simulink model "EMT_ML.before_diagnostic_fixes"  (R2024b)
settings: Solver=ode5  StartTime=0.0  StopTime=200  FixedStep=0.002  RelTol=1e-3
model workspace (MAT data in the model file):
  A = 7.3
  B = 2.71
  C0_shift = 200
  C1_shift = 200
  C2_shift = 200
  Cb = 70
  Cd = 0.6
  EMSInputBus : Simulink.Bus (value not decoded)
  Fb_max = 247500
  JA = 0.4
  JB = 0.4
  JZ = 0.4
  Jc1r2 = 0.01
  Jc3r4 = 0.01
  Jc4 = 0.01
  Je = 2.5
  Jh = 0.01
  Jq1 = 0.01
  Jq2 = 0.01
  Jr1 = 0.01
  Jr3s4 = 0.01
  Js123 = 0.01
  L = 4.472
  NE = [1600 1600 1600 1600 1600 1600 1600 1600 1600 1600 1600 1600 ... (840 elements, 30x28)]
  N_Te = 30
  N_ne = 28
  PE = [0 100.366530527 133.710336161 167.221698607 195.706356687 221.845219395 250.497434286 278.144308305 305.288511886 330.086920096 352.87464656 374.489475338 ... (840 elements, 30x28)]
  PN0 = 0
  Pb_epr = [-45 -45 -40 -30 0 30 40 45 45]
  Pb_max = [0 40 45 45 45]
  Pb_min = [-45 -45 -45 -40 0]
  Pe_ass = 230
  Pe_max = 1103
  Peg = [0 100 120 140 160 180 200 220 240 260 280 300 ... (53 elements, 1x53)]
  R_map = [0.09 0.089 0.09 0.091 0.092 0.093 0.094 0.095 0.096 0.097 0.098]
  SF_C0 = 1.5
  SF_C1 = 1.5
  SF_C2 = 1.5
  SF_Z1 = 1.5
  SF_Z2 = 1.5
  SF_ZD = 1.5
  SOC0 = 60
  SOC_epr = [30 31 50 59 60 61 70 79 80]
  SOC_map = [0 10 20 30 40 50 60 70 80 90 100]
  TA_max_map = [588.855 593.803361345 598.83559322 603.953846154 609.160344828 614.457391304 619.847368421 625.332743363 630.916071429 636.6 642.387272727 648.280733945 ... (115 elements, 1x115)]
  TA_min_map = [-588.855 -593.803361345 -598.83559322 -603.953846154 -609.160344828 -614.457391304 -619.847368421 -625.332743363 -630.916071429 -636.6 -642.387272727 -648.280733945 ... (115 elements, 1x115)]
  TAf = 0
  TB_max_map = [588.855 593.803361345 598.83559322 603.953846154 609.160344828 614.457391304 619.847368421 625.332743363 630.916071429 636.6 642.387272727 648.280733945 ... (115 elements, 1x115)]
  TB_min_map = [-588.855 -593.803361345 -598.83559322 -603.953846154 -609.160344828 -614.457391304 -619.847368421 -625.332743363 -630.916071429 -636.6 -642.387272727 -648.280733945 ... (115 elements, 1x115)]
  TBf = 0
  TE = [0 599 798 998 1168 1324 1495 1660 1822 1970 2106 2235 ... (840 elements, 30x28)]
  TS_A = 0.2
  TS_B = 0.2
  TS_C0 = 0.2
  TS_C1 = 0.2
  TS_C2 = 0.2
  TS_Z = 0.2
  TS_Z1 = 0.2
  TS_Z2 = 0.2
  TS_ZD = 0.2
  TZ_max_map = [537.13125 540.509433962 543.930379747 547.394904459 550.903846154 554.458064516 558.058441558 561.705882353 565.401315789 569.145695364 572.94 576.785234899 ... (131 elements, 1x131)]
  TZ_min_map = [-537.13125 -540.509433962 -543.930379747 -547.394904459 -550.903846154 -554.458064516 -558.058441558 -561.705882353 -565.401315789 -569.145695364 -572.94 -576.785234899 ... (131 elements, 1x131)]
  TZf = 0
  T_generator = [0 185 493.333333333 801.666666667 1110 1418.33333333 1726.66666667]
  T_motor = [0 185 493.333333333 801.666666667 1110 1418.33333333 1726.66666667]
  Te_map = [0 599 798 998 1168 1324 1495 1660 1822 1970 2106 2235 ... (30 elements, 1x30)]
  Te_max = 2754
  Te_max_map = [1168 1324 1495 1660 1822 1970 2106 2235 2355 2458 2543 2606 ... (28 elements, 1x28)]
  Te_start = 1600
  Tef = 100
  Teg = [0 596.8125 636.6 718.741935484 799.916230366 859.41 954.422788606 954.9 996.417391304 1078.98305085 1114.05 1169.26530612 ... (53 elements, 1x53)]
  Temax = 998
  Time = [0 0.1 0.2 0.3 0.4 0.5 0.6 0.7 0.8 0.9 1 1.1 ... (2001 elements, 1x2001)]
  Time_ele = [0 4 8 12 16 20 24 28 32 36 40 44 ... (401 elements, 1x401)]
  Time_fg = [0 2 4 6 8 10 12 14 16 18 20 22 ... (801 elements, 1x801)]
  Tmax_C0 = 2754
  Tmax_C1 = 3505.25455609
  Tmax_C2 = 3505.25455609
  Tmax_Z1 = 5584.80955498
  Tmax_Z2 = 16307.6439005
  Tmax_ZD = 3855.6
  Ts_e = 0.1
  Uoc_map = [814.5 917 933.25 945.75 958.25 969.25 978 985.25 993.25 1003.25 1050]
  V_Shift12 = 32
  V_Shift21 = 25
  V_Start = 10
  Voltage0 = 900
  Voltage_epr = [750 760 900 1000 1050]
  Y_engine = 0.955
  Yc = 0.98
  Yh = 0.96
  Yo = 0.92
  Yq = 0.94
  Z1_shift = 200
  Z2_shift = 200
  a11 = 1.54241568346
  a11_L = 1.54241568346
  a12 = -3.86074191629
  a12_L = 2.43173643789
  a21 = -1.04963112005
  a22 = 2.46948356808
  b11 = 0
  b11_L = 0
  b12 = 3.33
  b12_L = 7.8036
  b21 = 2.23571428571
  b22 = -2.13
  c11 = -0.648333656565
  c12 = 0
  c21 = -0.648333656565
  c22 = 0.680511182109
  controller_id = 1
  controller_name = 'Existing heuristic-grid EMS'
  cycle_grade = [0 0 0 0 0 0 0 0 0 0 0 0 ... (2001 elements, 1x2001)]
  cycle_road = [0.045 0.045 0.045 0.045 0.045 0.045 0.045 0.045 0.045 0.045 0.045 0.045 ... (2001 elements, 1x2001)]
  cycle_steering = [0 0 0 0 0 0 0 0 0 0 0 0 ... (2001 elements, 1x2001)]
  cycle_time = [0 0.1 0.2 0.3 0.4 0.5 0.6 0.7 0.8 0.9 1 1.1 ... (2001 elements, 1x2001)]
  d11 = -0.751666343435
  d12 = 0.3003003003
  d21 = -0.751666343435
  d22 = 0.319488817891
  e11 = -1.54241568346
  e12 = 0
  e21 = 1.04963112005
  e22 = -2.23571428571
  eff_generator = [0.8 0.8 0.79 0.79 0.76 0.74 0.72 0.8 0.85 0.88 0.85 0.8 ... (84 elements, 7x12)]
  eff_motor = [0.8 0.8 0.79 0.79 0.76 0.74 0.72 0.8 0.85 0.88 0.85 0.8 ... (84 elements, 7x12)]
  ele_map = [10 11.46 14.13 19.24 20.94 23.21 20.29 20.23 22.28 17.66 16.24 18.95 ... (401 elements, 1x401)]
  ems_runtime_config : object (value not decoded)
  f11 = -3.86074191629
  f12 = 3.33
  f21 = 2.46948356808
  f22 = -2.13
  fg = 0.045
  fg_map = [0.0125 0.0215 0.0332 0.0452 0.0525 0.0589 0.0584 0.0592 0.0621 0.0576 0.055 0.0572 ... (801 elements, 1x801)]
  fuel_gpkwh = [269.874826377 269.874826377 260.084605263 254.895150301 249.802821062 244.062054381 234.972466555 226.630558735 223.93243551 227.612775381 231.379615385 228.983738255 ... (840 elements, 30x28)]
  fuel_map = [269.874826377 269.874826377 260.084605263 254.895150301 249.802821062 244.062054381 234.972466555 226.630558735 223.93243551 227.612775381 231.379615385 228.983738255 ... (840 elements, 30x28)]
  fuel_map_N = [269.874826377 269.874826377 260.084605263 254.895150301 249.802821062 nan nan nan nan nan nan nan ... (840 elements, 30x28)]
  i = 28
  ic = 4.42
  iq = 1.4
  it = 4
  j = 30
  k1 = 2.13
  k2 = 2.13
  k3 = 2.33
  k4 = 1.92
  kh = 2.88
  kq = 2.17
  kt = 1.83
  mass = 45000
  miu_max = 0.8
  nA_map = [-6000 -5950 -5900 -5850 -5800 -5750 -5700 -5650 -5600 -5550 -5500 -5450 ... (115 elements, 1x115)]
  nA_max = 6000
  nA_min = -6000
  nB_map = [-6000 -5950 -5900 -5850 -5800 -5750 -5700 -5650 -5600 -5550 -5500 -5450 ... (115 elements, 1x115)]
  nB_max = 6000
  nB_min = -6000
  nB_start = 0
  nZ_map = [-8000 -7950 -7900 -7850 -7800 -7750 -7700 -7650 -7600 -7550 -7500 -7450 ... (131 elements, 1x131)]
  nZ_max = 8000
  nZ_min = -8000
  n_generator = [0 318.5 796.25 1274 1751.75 2229.5 2707.25 3185 3662.75 4140.5 4618.25 7007]
  n_motor = [0 318.5 796.25 1274 1751.75 2229.5 2707.25 3185 3662.75 4140.5 4618.25 7007]
  ne_idl = 3000
  ne_map = [1600 1700 1800 1900 2000 2100 2200 2300 2400 2500 2600 2700 ... (28 elements, 1x28)]
  ne_max = 4200
  ne_min = 1600
  ne_start = 200
  neg = [1600 1600 1800 1860 1910 2000 2001 2200 2300 2301 2400 2450 ... (53 elements, 1x53)]
  no_Shift12 = 1589.43589002
  no_Shift21 = 1241.74678908
  rz = 0.318
  startup_feedback_delay_s = 0.002
  startup_power_share = 0.5
  startup_speed_regularizer_rpm = 100
  v_cyc = [0 0 0 0 0 0 0 0 0 0 0 0 ... (2001 elements, 1x2001)]
  voltage_HighA = 1050
  voltage_HighB = 1050
  voltage_HighZ = 1050
  voltage_LowA = 750
  voltage_LowB = 750
  voltage_LowZ = 750
symbols that are objects in the model workspace (value not decoded): ems_runtime_config
undefined symbols (not defined in the file or in its folder): sigbuilder_block
libraries: fl_lib x82, nesl_utility x55, simulink x49, sdl_lib x10, simulink_need_slupdate x6, powerlib_extras x1
(part 6 of 7)

== system EMT_ML.before_diagnostic_fixes/Control Unit/Control/Shift Stage/EVT2->EVT1/engine torque ==
  Te_com : Outport
  wires:
  [Te_ref] -> Te_com/1

== system EMT_ML.before_diagnostic_fixes/Control Unit/Control/Shift Stage/EVT2->EVT1/motorA torque ==
  TA_com : Outport
  wires:
  [TA_ref] -> TA_com/1

== system EMT_ML.before_diagnostic_fixes/Control Unit/Control/Shift Stage/EVT2->EVT1/motorB torque ==
  TB_com : Outport
  wires:
  [TB_ref] -> TB_com/1

== system EMT_ML.before_diagnostic_fixes/Control Unit/Control/Shift Stage/EVT2->EVT1/motorZ torque ==
  Lookup Table : Lookup  InputValues=nZ_map  Table=TZ_max_map  SaturateOnIntegerOverflow=off
  Lookup Table1 : Lookup  InputValues=nZ_map  Table=TZ_min_map  SaturateOnIntegerOverflow=off
  Saturation Dynamic : simulink/Discontinuities/Saturation Dynamic  OutMin=[]  OutMax=[]  OutDataTypeStr=Inherit: Same as second input  OutDataType=sfix(16)  OutScaling=2^-10  DoSatur=off
  Saturation1 : Saturate  UpperLimit=max(nZ_map)  LowerLimit=min(nZ_map)
  Saturation2 : Saturate  UpperLimit=max(nZ_map)  LowerLimit=min(nZ_map)
  Subsystem1 : Subsystem
  TZ_com : Outport
  wires:
  Saturation Dynamic/1 -> TZ_com/1
  [nZ_act] -> Saturation1/1, Saturation2/1, Subsystem1/1(nZ_act)
  Lookup Table/1 -> Saturation Dynamic/1
  Lookup Table1/1 -> Saturation Dynamic/3
  Saturation1/1 -> Lookup Table/1
  Saturation2/1 -> Lookup Table1/1
  Subsystem1/1(TZ_com) -> Saturation Dynamic/2

== system EMT_ML.before_diagnostic_fixes/Control Unit/Driver/Electric Power Requirement/Subsystem4/Subsystem4 ==
  11 : Constant
  21 : Constant  Value=2
  22 : Constant  Value=3
  31 : Constant  Value=4
  0.1 : Outport
  0.01 : Outport  Port=2
  10 : Outport  Port=3
  100 : Outport  Port=4
  wires:
  31/1 -> 100/1
  22/1 -> 10/1
  21/1 -> 0.01/1
  11/1 -> 0.1/1

== system EMT_ML.before_diagnostic_fixes/Control Unit/Driver/Electric Power Requirement/Subsystem4/Subsystem6 ==
  11 : Constant
  21 : Constant  Value=2
  22 : Constant  Value=3
  31 : Constant  Value=4
  1 : Outport
  2 : Outport  Port=2
  3 : Outport  Port=3
  4 : Outport  Port=4
  wires:
  11/1 -> 1/1
  21/1 -> 2/1
  22/1 -> 3/1
  31/1 -> 4/1

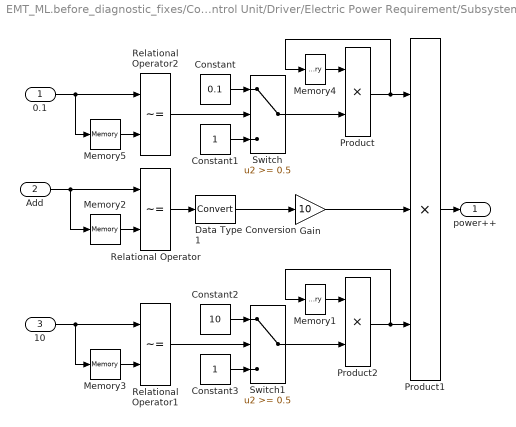
== system EMT_ML.before_diagnostic_fixes/Control Unit/Driver/Electric Power Requirement/Subsystem6/Subsystem ==
  0.1 : Inport
  Add : Inport  Port=2
  10 : Inport  Port=3
  Constant : Constant  Value=0.1
  Constant1 : Constant
  Constant2 : Constant  Value=10
  Constant3 : Constant
  Data Type Conversion1 : DataTypeConversion  SaturateOnIntegerOverflow=off  RndMeth=Floor
  Gain : Gain  Gain=10
  Memory1 : Memory  InitialCondition=1
  Memory2 : Memory
  Memory3 : Memory
  Memory4 : Memory  InitialCondition=1
  Memory5 : Memory
  Product : Product  RndMeth=Zero
  Product1 : Product  Inputs=3  RndMeth=Zero
  Product2 : Product  RndMeth=Zero
  Relational Operator : RelationalOperator  Operator=~=  OutDataTypeStr=boolean  InputSameDT=off
  Relational Operator1 : RelationalOperator  Operator=~=  OutDataTypeStr=boolean  InputSameDT=off
  Relational Operator2 : RelationalOperator  Operator=~=  OutDataTypeStr=boolean  InputSameDT=off
  Switch : Switch  Threshold=0.5  SaturateOnIntegerOverflow=off  InputSameDT=off
  Switch1 : Switch  Threshold=0.5  SaturateOnIntegerOverflow=off  InputSameDT=off
  power++ : Outport
  wires:
  Memory2/1 -> Relational Operator/2
  Add/1 -> Relational Operator/1, Memory2/1
  Relational Operator/1 -> Data Type Conversion1/1
  Data Type Conversion1/1 -> Gain/1
  Product/1 -> Memory4/1, Product1/1
  Memory4/1 -> Product/1
  Memory5/1 -> Relational Operator2/2
  Relational Operator2/1 -> Switch/2
  0.1/1 -> Memory5/1, Relational Operator2/1
  Constant/1 -> Switch/1
  Constant1/1 -> Switch/3
  Switch/1 -> Product/2
  Product1/1 -> power++/1
  Product2/1 -> Memory1/1, Product1/3
  Memory1/1 -> Product2/1
  Memory3/1 -> Relational Operator1/2
  Relational Operator1/1 -> Switch1/2
  10/1 -> Relational Operator1/1, Memory3/1
  Constant2/1 -> Switch1/1
  Constant3/1 -> Switch1/3
  Switch1/1 -> Product2/2
  Gain/1 -> Product1/2

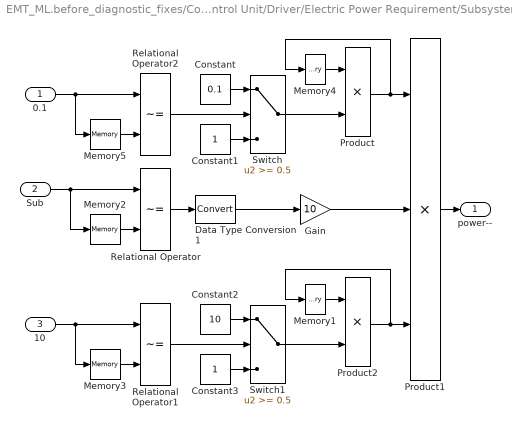
== system EMT_ML.before_diagnostic_fixes/Control Unit/Driver/Electric Power Requirement/Subsystem6/Subsystem1 ==
  0.1 : Inport
  Sub : Inport  Port=2
  10 : Inport  Port=3
  Constant : Constant  Value=0.1
  Constant1 : Constant
  Constant2 : Constant  Value=10
  Constant3 : Constant
  Data Type Conversion1 : DataTypeConversion  SaturateOnIntegerOverflow=off  RndMeth=Floor
  Gain : Gain  Gain=10
  Memory1 : Memory  InitialCondition=1
  Memory2 : Memory
  Memory3 : Memory
  Memory4 : Memory  InitialCondition=1
  Memory5 : Memory
  Product : Product  RndMeth=Zero
  Product1 : Product  Inputs=3  RndMeth=Zero
  Product2 : Product  RndMeth=Zero
  Relational Operator : RelationalOperator  Operator=~=  OutDataTypeStr=boolean  InputSameDT=off
  Relational Operator1 : RelationalOperator  Operator=~=  OutDataTypeStr=boolean  InputSameDT=off
  Relational Operator2 : RelationalOperator  Operator=~=  OutDataTypeStr=boolean  InputSameDT=off
  Switch : Switch  Threshold=0.5  SaturateOnIntegerOverflow=off  InputSameDT=off
  Switch1 : Switch  Threshold=0.5  SaturateOnIntegerOverflow=off  InputSameDT=off
  power-- : Outport
  wires:
  Switch1/1 -> Product2/2
  Constant3/1 -> Switch1/3
  Constant2/1 -> Switch1/1
  10/1 -> Memory3/1, Relational Operator1/1
  Relational Operator1/1 -> Switch1/2
  Memory3/1 -> Relational Operator1/2
  Memory1/1 -> Product2/1
  Product2/1 -> Product1/3, Memory1/1
  Product1/1 -> power--/1
  Switch/1 -> Product/2
  Constant1/1 -> Switch/3
  Constant/1 -> Switch/1
  0.1/1 -> Relational Operator2/1, Memory5/1
  Relational Operator2/1 -> Switch/2
  Memory5/1 -> Relational Operator2/2
  Memory4/1 -> Product/1
  Product/1 -> Product1/1, Memory4/1
  Data Type Conversion1/1 -> Gain/1
  Relational Operator/1 -> Data Type Conversion1/1
  Sub/1 -> Memory2/1, Relational Operator/1
  Memory2/1 -> Relational Operator/2
  Gain/1 -> Product1/2

== system EMT_ML.before_diagnostic_fixes/Control Unit/Driver/Grade Angle/Subsystem4/Subsystem4 ==
  11 : Constant
  21 : Constant  Value=2
  22 : Constant  Value=3
  31 : Constant  Value=4
  0.1 : Outport
  0.01 : Outport  Port=2
  10 : Outport  Port=3
  100 : Outport  Port=4
  wires:
  31/1 -> 100/1
  22/1 -> 10/1
  21/1 -> 0.01/1
  11/1 -> 0.1/1

== system EMT_ML.before_diagnostic_fixes/Control Unit/Driver/Grade Angle/Subsystem4/Subsystem6 ==
  11 : Constant
  21 : Constant  Value=2
  22 : Constant  Value=3
  31 : Constant  Value=4
  1 : Outport
  2 : Outport  Port=2
  3 : Outport  Port=3
  4 : Outport  Port=4
  wires:
  11/1 -> 1/1
  21/1 -> 2/1
  22/1 -> 3/1
  31/1 -> 4/1

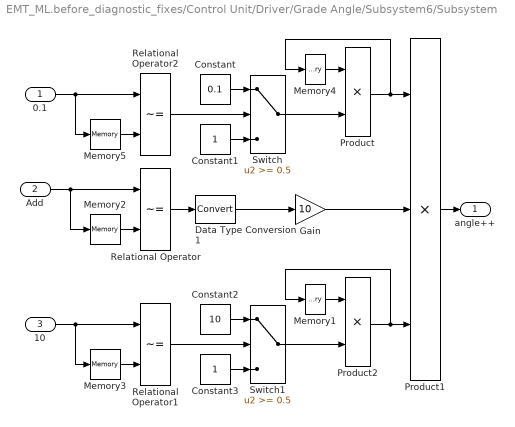
== system EMT_ML.before_diagnostic_fixes/Control Unit/Driver/Grade Angle/Subsystem6/Subsystem ==
  0.1 : Inport
  Add : Inport  Port=2
  10 : Inport  Port=3
  Constant : Constant  Value=0.1
  Constant1 : Constant
  Constant2 : Constant  Value=10
  Constant3 : Constant
  Data Type Conversion1 : DataTypeConversion  SaturateOnIntegerOverflow=off  RndMeth=Floor
  Gain : Gain  Gain=10
  Memory1 : Memory  InitialCondition=1
  Memory2 : Memory
  Memory3 : Memory
  Memory4 : Memory  InitialCondition=1
  Memory5 : Memory
  Product : Product  RndMeth=Zero
  Product1 : Product  Inputs=3  RndMeth=Zero
  Product2 : Product  RndMeth=Zero
  Relational Operator : RelationalOperator  Operator=~=  OutDataTypeStr=boolean  InputSameDT=off
  Relational Operator1 : RelationalOperator  Operator=~=  OutDataTypeStr=boolean  InputSameDT=off
  Relational Operator2 : RelationalOperator  Operator=~=  OutDataTypeStr=boolean  InputSameDT=off
  Switch : Switch  Threshold=0.5  SaturateOnIntegerOverflow=off  InputSameDT=off
  Switch1 : Switch  Threshold=0.5  SaturateOnIntegerOverflow=off  InputSameDT=off
  angle++ : Outport
  wires:
  Memory2/1 -> Relational Operator/2
  Add/1 -> Relational Operator/1, Memory2/1
  Relational Operator/1 -> Data Type Conversion1/1
  Data Type Conversion1/1 -> Gain/1
  Product/1 -> Memory4/1, Product1/1
  Memory4/1 -> Product/1
  Memory5/1 -> Relational Operator2/2
  Relational Operator2/1 -> Switch/2
  0.1/1 -> Memory5/1, Relational Operator2/1
  Constant/1 -> Switch/1
  Constant1/1 -> Switch/3
  Switch/1 -> Product/2
  Product1/1 -> angle++/1
  Product2/1 -> Memory1/1, Product1/3
  Memory1/1 -> Product2/1
  Memory3/1 -> Relational Operator1/2
  Relational Operator1/1 -> Switch1/2
  10/1 -> Relational Operator1/1, Memory3/1
  Constant2/1 -> Switch1/1
  Constant3/1 -> Switch1/3
  Switch1/1 -> Product2/2
  Gain/1 -> Product1/2

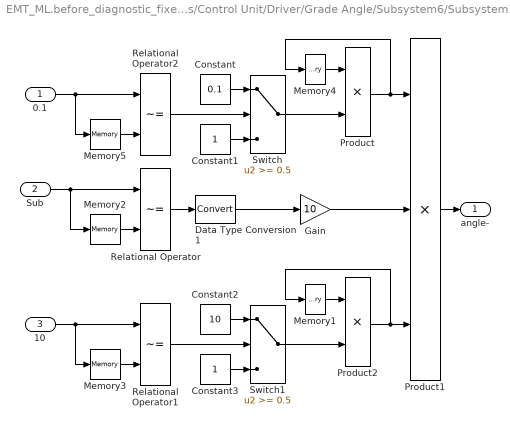
== system EMT_ML.before_diagnostic_fixes/Control Unit/Driver/Grade Angle/Subsystem6/Subsystem1 ==
  0.1 : Inport
  Sub : Inport  Port=2
  10 : Inport  Port=3
  Constant : Constant  Value=0.1
  Constant1 : Constant
  Constant2 : Constant  Value=10
  Constant3 : Constant
  Data Type Conversion1 : DataTypeConversion  SaturateOnIntegerOverflow=off  RndMeth=Floor
  Gain : Gain  Gain=10
  Memory1 : Memory  InitialCondition=1
  Memory2 : Memory
  Memory3 : Memory
  Memory4 : Memory  InitialCondition=1
  Memory5 : Memory
  Product : Product  RndMeth=Zero
  Product1 : Product  Inputs=3  RndMeth=Zero
  Product2 : Product  RndMeth=Zero
  Relational Operator : RelationalOperator  Operator=~=  OutDataTypeStr=boolean  InputSameDT=off
  Relational Operator1 : RelationalOperator  Operator=~=  OutDataTypeStr=boolean  InputSameDT=off
  Relational Operator2 : RelationalOperator  Operator=~=  OutDataTypeStr=boolean  InputSameDT=off
  Switch : Switch  Threshold=0.5  SaturateOnIntegerOverflow=off  InputSameDT=off
  Switch1 : Switch  Threshold=0.5  SaturateOnIntegerOverflow=off  InputSameDT=off
  angle- : Outport
  wires:
  Switch1/1 -> Product2/2
  Constant3/1 -> Switch1/3
  Constant2/1 -> Switch1/1
  10/1 -> Memory3/1, Relational Operator1/1
  Relational Operator1/1 -> Switch1/2
  Memory3/1 -> Relational Operator1/2
  Memory1/1 -> Product2/1
  Product2/1 -> Product1/3, Memory1/1
  Product1/1 -> angle-/1
  Switch/1 -> Product/2
  Constant1/1 -> Switch/3
  Constant/1 -> Switch/1
  0.1/1 -> Relational Operator2/1, Memory5/1
  Relational Operator2/1 -> Switch/2
  Memory5/1 -> Relational Operator2/2
  Memory4/1 -> Product/1
  Product/1 -> Product1/1, Memory4/1
  Data Type Conversion1/1 -> Gain/1
  Relational Operator/1 -> Data Type Conversion1/1
  Sub/1 -> Memory2/1, Relational Operator/1
  Memory2/1 -> Relational Operator/2
  Gain/1 -> Product1/2

== system EMT_ML.before_diagnostic_fixes/Control Unit/Driver/Ground Resistance Coefficient/Road/Subsystem ==
  In : Inport
  Add : Sum  Inputs=+++
  Compare To Constant1 : simulink/Logic and Bit Operations/Compare To Constant  relop=>  const=0.01  OutDataTypeStr=uint8
  Compare To Constant2 : simulink/Logic and Bit Operations/Compare To Constant  relop=>  const=0.2  OutDataTypeStr=uint8
  Compare To Constant3 : simulink/Logic and Bit Operations/Compare To Constant  relop=>  const=0.8  OutDataTypeStr=uint8
  Compare To Constant4 : simulink/Logic and Bit Operations/Compare To Constant  relop=<  const=1  OutDataTypeStr=uint8
  Data Type Conversion : DataTypeConversion  SaturateOnIntegerOverflow=off  RndMeth=Floor
  Logical Operator1 : Logic  Operator=OR  AllPortsSameDT=off  OutDataTypeStr=boolean
  Memory2 : Memory
  Judge : Outport
  wires:
  Compare To Constant2/1 -> Add/2
  Data Type Conversion/1 -> Judge/1
  Compare To Constant1/1 -> Add/1
  Add/1 -> Data Type Conversion/1
  In/1 -> Compare To Constant3/1, Compare To Constant2/1, Compare To Constant1/1
  [v_act] -> Memory2/1
  Memory2/1 -> Compare To Constant4/1
  Compare To Constant4/1 -> Logical Operator1/2
  Compare To Constant3/1 -> Logical Operator1/1
  Logical Operator1/1 -> Add/3

== system EMT_ML.before_diagnostic_fixes/Control Unit/Driver/Ground Resistance Coefficient/Road/Subsystem1 ==
  Constant5 : Constant  Value=0.6
  Out1 : Outport
  wires:
  Constant5/1 -> Out1/1

== system EMT_ML.before_diagnostic_fixes/Control Unit/Driver/Ground Resistance Coefficient/Road/Subsystem2 ==
  In1 : Inport
  1-D Lookup Table : Lookup_n-D  NumberOfTableDimensions=1  BreakpointsForDimension1=[-1 0 0.1 0.2 0.8 1]  Table=[0.6 0.1 0.04 0 0 0]  RndMeth=Simplest
  Saturation : Saturate  UpperLimit=1  LowerLimit=-1
  Out1 : Outport
  wires:
  Saturation/1 -> 1-D Lookup Table/1
  In1/1 -> Saturation/1
  1-D Lookup Table/1 -> Out1/1

== system EMT_ML.before_diagnostic_fixes/Control Unit/Driver/Ground Resistance Coefficient/Road/Subsystem3 ==
  Constant1 : Constant  Value=0
  Out1 : Outport
  wires:
  Constant1/1 -> Out1/1

== system EMT_ML.before_diagnostic_fixes/Control Unit/Driver/Ground Resistance Coefficient/Road/Subsystem4 ==
  Constant1 : Constant  Value=-0.04
  Out1 : Outport
  wires:
  Constant1/1 -> Out1/1

== system EMT_ML.before_diagnostic_fixes/Control Unit/Driver/Ground Resistance Coefficient/Subsystem2/Subsystem4 ==
  11 : Constant
  21 : Constant  Value=2
  22 : Constant  Value=3
  31 : Constant  Value=4
  0.1 : Outport
  0.01 : Outport  Port=2
  10 : Outport  Port=3
  100 : Outport  Port=4
  wires:
  11/1 -> 0.1/1
  21/1 -> 0.01/1
  22/1 -> 10/1
  31/1 -> 100/1

== system EMT_ML.before_diagnostic_fixes/Control Unit/Driver/Ground Resistance Coefficient/Subsystem2/Subsystem6 ==
  11 : Constant
  21 : Constant  Value=2
  22 : Constant  Value=3
  31 : Constant  Value=4
  1 : Outport
  2 : Outport  Port=2
  3 : Outport  Port=3
  4 : Outport  Port=4
  wires:
  31/1 -> 4/1
  22/1 -> 3/1
  21/1 -> 2/1
  11/1 -> 1/1

== system EMT_ML.before_diagnostic_fixes/Control Unit/Driver/Ground Resistance Coefficient/Subsystem3/Subsystem ==
  0.1 : Inport
  Add : Inport  Port=2
  10 : Inport  Port=3
  Constant : Constant  Value=0.1
  Constant1 : Constant
  Constant2 : Constant  Value=10
  Constant3 : Constant
  Data Type Conversion1 : DataTypeConversion  SaturateOnIntegerOverflow=off  RndMeth=Floor
  Gain : Gain  Gain=0.01
  Memory1 : Memory  InitialCondition=1
  Memory2 : Memory
  Memory3 : Memory
  Memory4 : Memory  InitialCondition=1
  Memory5 : Memory
  Product : Product  RndMeth=Zero
  Product1 : Product  Inputs=3  RndMeth=Zero
  Product2 : Product  RndMeth=Zero
  Relational Operator : RelationalOperator  Operator=~=  OutDataTypeStr=boolean  InputSameDT=off
  Relational Operator1 : RelationalOperator  Operator=~=  OutDataTypeStr=boolean  InputSameDT=off
  Relational Operator2 : RelationalOperator  Operator=~=  OutDataTypeStr=boolean  InputSameDT=off
  Switch : Switch  Threshold=0.5  SaturateOnIntegerOverflow=off  InputSameDT=off
  Switch1 : Switch  Threshold=0.5  SaturateOnIntegerOverflow=off  InputSameDT=off
  fg++ : Outport
  wires:
  Gain/1 -> Product1/2
  Switch1/1 -> Product2/2
  Constant3/1 -> Switch1/3
  Constant2/1 -> Switch1/1
  10/1 -> Memory3/1, Relational Operator1/1
  Relational Operator1/1 -> Switch1/2
  Memory3/1 -> Relational Operator1/2
  Memory1/1 -> Product2/1
  Product2/1 -> Product1/3, Memory1/1
  Product1/1 -> fg++/1
  Switch/1 -> Product/2
  Constant1/1 -> Switch/3
  Constant/1 -> Switch/1
  0.1/1 -> Relational Operator2/1, Memory5/1
  Relational Operator2/1 -> Switch/2
  Memory5/1 -> Relational Operator2/2
  Memory4/1 -> Product/1
  Product/1 -> Product1/1, Memory4/1
  Data Type Conversion1/1 -> Gain/1
  Relational Operator/1 -> Data Type Conversion1/1
  Add/1 -> Memory2/1, Relational Operator/1
  Memory2/1 -> Relational Operator/2

== system EMT_ML.before_diagnostic_fixes/Control Unit/Driver/Ground Resistance Coefficient/Subsystem3/Subsystem1 ==
  0.1 : Inport
  Sub : Inport  Port=2
  10 : Inport  Port=3
  Constant : Constant  Value=0.1
  Constant1 : Constant
  Constant2 : Constant  Value=10
  Constant3 : Constant
  Data Type Conversion1 : DataTypeConversion  SaturateOnIntegerOverflow=off  RndMeth=Floor
  Gain : Gain  Gain=0.01
  Memory1 : Memory  InitialCondition=1
  Memory2 : Memory
  Memory3 : Memory
  Memory4 : Memory  InitialCondition=1
  Memory5 : Memory
  Product : Product  RndMeth=Zero
  Product1 : Product  Inputs=3  RndMeth=Zero
  Product2 : Product  RndMeth=Zero
  Relational Operator : RelationalOperator  Operator=~=  OutDataTypeStr=boolean  InputSameDT=off
  Relational Operator1 : RelationalOperator  Operator=~=  OutDataTypeStr=boolean  InputSameDT=off
  Relational Operator2 : RelationalOperator  Operator=~=  OutDataTypeStr=boolean  InputSameDT=off
  Switch : Switch  Threshold=0.5  SaturateOnIntegerOverflow=off  InputSameDT=off
  Switch1 : Switch  Threshold=0.5  SaturateOnIntegerOverflow=off  InputSameDT=off
  fg-- : Outport
  wires:
  Gain/1 -> Product1/2
  Memory2/1 -> Relational Operator/2
  Sub/1 -> Relational Operator/1, Memory2/1
  Relational Operator/1 -> Data Type Conversion1/1
  Data Type Conversion1/1 -> Gain/1
  Product/1 -> Memory4/1, Product1/1
  Memory4/1 -> Product/1
  Memory5/1 -> Relational Operator2/2
  Relational Operator2/1 -> Switch/2
  0.1/1 -> Memory5/1, Relational Operator2/1
  Constant/1 -> Switch/1
  Constant1/1 -> Switch/3
  Switch/1 -> Product/2
  Product1/1 -> fg--/1
  Product2/1 -> Memory1/1, Product1/3
  Memory1/1 -> Product2/1
  Memory3/1 -> Relational Operator1/2
  Relational Operator1/1 -> Switch1/2
  10/1 -> Relational Operator1/1, Memory3/1
  Constant2/1 -> Switch1/1
  Constant3/1 -> Switch1/3
  Switch1/1 -> Product2/2

== system EMT_ML.before_diagnostic_fixes/Control Unit/Driver/Pedal /Subsystem13/Subsystem4 ==
  11 : Constant
  21 : Constant  Value=2
  22 : Constant  Value=3
  31 : Constant  Value=4
  0.1 : Outport
  0.01 : Outport  Port=2
  10 : Outport  Port=3
  100 : Outport  Port=4
  wires:
  31/1 -> 100/1
  22/1 -> 10/1
  21/1 -> 0.01/1
  11/1 -> 0.1/1

== system EMT_ML.before_diagnostic_fixes/Control Unit/Driver/Pedal /Subsystem13/Subsystem6 ==
  11 : Constant
  21 : Constant  Value=2
  22 : Constant  Value=3
  31 : Constant  Value=4
  1 : Outport
  2 : Outport  Port=2
  3 : Outport  Port=3
  4 : Outport  Port=4
  wires:
  11/1 -> 1/1
  21/1 -> 2/1
  22/1 -> 3/1
  31/1 -> 4/1

== system EMT_ML.before_diagnostic_fixes/Control Unit/Driver/Pedal /Subsystem5/Subsystem ==
  0.1 : Inport
  Add : Inport  Port=2
  10 : Inport  Port=3
  Constant : Constant  Value=0.1
  Constant1 : Constant
  Constant2 : Constant  Value=10
  Constant3 : Constant
  Data Type Conversion1 : DataTypeConversion  SaturateOnIntegerOverflow=off  RndMeth=Floor
  Gain : Gain  Gain=0.1
  Memory1 : Memory  InitialCondition=1
  Memory2 : Memory
  Memory3 : Memory
  Memory4 : Memory  InitialCondition=1
  Memory5 : Memory
  Product : Product  RndMeth=Zero
  Product1 : Product  Inputs=3  RndMeth=Zero
  Product2 : Product  RndMeth=Zero
  Relational Operator : RelationalOperator  Operator=~=  OutDataTypeStr=boolean  InputSameDT=off
  Relational Operator1 : RelationalOperator  Operator=~=  OutDataTypeStr=boolean  InputSameDT=off
  Relational Operator2 : RelationalOperator  Operator=~=  OutDataTypeStr=boolean  InputSameDT=off
  Switch : Switch  Threshold=0.5  SaturateOnIntegerOverflow=off  InputSameDT=off
  Switch1 : Switch  Threshold=0.5  SaturateOnIntegerOverflow=off  InputSameDT=off
  pedal++ : Outport
  wires:
  Memory2/1 -> Relational Operator/2
  Add/1 -> Relational Operator/1, Memory2/1
  Relational Operator/1 -> Data Type Conversion1/1
  Data Type Conversion1/1 -> Gain/1
  Product/1 -> Memory4/1, Product1/1
  Memory4/1 -> Product/1
  Memory5/1 -> Relational Operator2/2
  Relational Operator2/1 -> Switch/2
  0.1/1 -> Memory5/1, Relational Operator2/1
  Constant/1 -> Switch/1
  Constant1/1 -> Switch/3
  Switch/1 -> Product/2
  Product1/1 -> pedal++/1
  Product2/1 -> Memory1/1, Product1/3
  Memory1/1 -> Product2/1
  Memory3/1 -> Relational Operator1/2
  Relational Operator1/1 -> Switch1/2
  10/1 -> Relational Operator1/1, Memory3/1
  Constant2/1 -> Switch1/1
  Constant3/1 -> Switch1/3
  Switch1/1 -> Product2/2
  Gain/1 -> Product1/2

== system EMT_ML.before_diagnostic_fixes/Control Unit/Driver/Pedal /Subsystem5/Subsystem1 ==
  0.1 : Inport
  Sub : Inport  Port=2
  10 : Inport  Port=3
  Constant : Constant  Value=0.1
  Constant1 : Constant
  Constant2 : Constant  Value=10
  Constant3 : Constant
  Data Type Conversion1 : DataTypeConversion  SaturateOnIntegerOverflow=off  RndMeth=Floor
  Gain : Gain  Gain=0.1
  Memory1 : Memory  InitialCondition=1
  Memory2 : Memory
  Memory3 : Memory
  Memory4 : Memory  InitialCondition=1
  Memory5 : Memory
  Product : Product  RndMeth=Zero
  Product1 : Product  Inputs=3  RndMeth=Zero
  Product2 : Product  RndMeth=Zero
  Relational Operator : RelationalOperator  Operator=~=  OutDataTypeStr=boolean  InputSameDT=off
  Relational Operator1 : RelationalOperator  Operator=~=  OutDataTypeStr=boolean  InputSameDT=off
  Relational Operator2 : RelationalOperator  Operator=~=  OutDataTypeStr=boolean  InputSameDT=off
  Switch : Switch  Threshold=0.5  SaturateOnIntegerOverflow=off  InputSameDT=off
  Switch1 : Switch  Threshold=0.5  SaturateOnIntegerOverflow=off  InputSameDT=off
  pedal-- : Outport
  wires:
  Switch1/1 -> Product2/2
  Constant3/1 -> Switch1/3
  Constant2/1 -> Switch1/1
  10/1 -> Memory3/1, Relational Operator1/1
  Relational Operator1/1 -> Switch1/2
  Memory3/1 -> Relational Operator1/2
  Memory1/1 -> Product2/1
  Product2/1 -> Product1/3, Memory1/1
  Product1/1 -> pedal--/1
  Switch/1 -> Product/2
  Constant1/1 -> Switch/3
  Constant/1 -> Switch/1
  0.1/1 -> Relational Operator2/1, Memory5/1
  Relational Operator2/1 -> Switch/2
  Memory5/1 -> Relational Operator2/2
  Memory4/1 -> Product/1
  Product/1 -> Product1/1, Memory4/1
  Data Type Conversion1/1 -> Gain/1
  Relational Operator/1 -> Data Type Conversion1/1
  Sub/1 -> Memory2/1, Relational Operator/1
  Memory2/1 -> Relational Operator/2
  Gain/1 -> Product1/2

== system EMT_ML.before_diagnostic_fixes/Control Unit/Driver/Wheel Angle/Subsystem1/Subsystem4 ==
  11 : Constant
  21 : Constant  Value=2
  22 : Constant  Value=3
  31 : Constant  Value=4
  0.1 : Outport
  0.01 : Outport  Port=2
  10 : Outport  Port=3
  100 : Outport  Port=4
  wires:
  31/1 -> 100/1
  22/1 -> 10/1
  21/1 -> 0.01/1
  11/1 -> 0.1/1

== system EMT_ML.before_diagnostic_fixes/Control Unit/Driver/Wheel Angle/Subsystem1/Subsystem6 ==
  11 : Constant
  21 : Constant  Value=2
  22 : Constant  Value=3
  31 : Constant  Value=4
  1 : Outport
  2 : Outport  Port=2
  3 : Outport  Port=3
  4 : Outport  Port=4
  wires:
  11/1 -> 1/1
  21/1 -> 2/1
  22/1 -> 3/1
  31/1 -> 4/1

== system EMT_ML.before_diagnostic_fixes/Control Unit/Driver/Wheel Angle/Subsystem2/Subsystem ==
  0.1 : Inport
  Add : Inport  Port=2
  10 : Inport  Port=3
  Constant : Constant  Value=0.1
  Constant1 : Constant
  Constant2 : Constant  Value=10
  Constant3 : Constant
  Data Type Conversion1 : DataTypeConversion  SaturateOnIntegerOverflow=off  RndMeth=Floor
  Gain : Gain
  Memory1 : Memory  InitialCondition=1
  Memory2 : Memory
  Memory3 : Memory
  Memory4 : Memory  InitialCondition=1
  Memory5 : Memory
  Product : Product  RndMeth=Zero
  Product1 : Product  Inputs=3  RndMeth=Zero
  Product2 : Product  RndMeth=Zero
  Relational Operator : RelationalOperator  Operator=~=  OutDataTypeStr=boolean  InputSameDT=off
  Relational Operator1 : RelationalOperator  Operator=~=  OutDataTypeStr=boolean  InputSameDT=off
  Relational Operator2 : RelationalOperator  Operator=~=  OutDataTypeStr=boolean  InputSameDT=off
  Switch : Switch  Threshold=0.5  SaturateOnIntegerOverflow=off  InputSameDT=off
  Switch1 : Switch  Threshold=0.5  SaturateOnIntegerOverflow=off  InputSameDT=off
  wheel++ : Outport
  wires:
  Memory2/1 -> Relational Operator/2
  Add/1 -> Relational Operator/1, Memory2/1
  Relational Operator/1 -> Data Type Conversion1/1
  Data Type Conversion1/1 -> Gain/1
  Product/1 -> Memory4/1, Product1/1
  Memory4/1 -> Product/1
  Memory5/1 -> Relational Operator2/2
  Relational Operator2/1 -> Switch/2
  0.1/1 -> Memory5/1, Relational Operator2/1
  Constant/1 -> Switch/1
  Constant1/1 -> Switch/3
  Switch/1 -> Product/2
  Product1/1 -> wheel++/1
  Product2/1 -> Memory1/1, Product1/3
  Memory1/1 -> Product2/1
  Memory3/1 -> Relational Operator1/2
  Relational Operator1/1 -> Switch1/2
  10/1 -> Relational Operator1/1, Memory3/1
  Constant2/1 -> Switch1/1
  Constant3/1 -> Switch1/3
  Switch1/1 -> Product2/2
  Gain/1 -> Product1/2

== system EMT_ML.before_diagnostic_fixes/Control Unit/Driver/Wheel Angle/Subsystem2/Subsystem1 ==
  0.1 : Inport
  Sub : Inport  Port=2
  10 : Inport  Port=3
  Constant : Constant  Value=0.1
  Constant1 : Constant
  Constant2 : Constant  Value=10
  Constant3 : Constant
  Data Type Conversion1 : DataTypeConversion  SaturateOnIntegerOverflow=off  RndMeth=Floor
  Gain : Gain
  Memory1 : Memory  InitialCondition=1
  Memory2 : Memory
  Memory3 : Memory
  Memory4 : Memory  InitialCondition=1
  Memory5 : Memory
  Product : Product  RndMeth=Zero
  Product1 : Product  Inputs=3  RndMeth=Zero
  Product2 : Product  RndMeth=Zero
  Relational Operator : RelationalOperator  Operator=~=  OutDataTypeStr=boolean  InputSameDT=off
  Relational Operator1 : RelationalOperator  Operator=~=  OutDataTypeStr=boolean  InputSameDT=off
  Relational Operator2 : RelationalOperator  Operator=~=  OutDataTypeStr=boolean  InputSameDT=off
  Switch : Switch  Threshold=0.5  SaturateOnIntegerOverflow=off  InputSameDT=off
  Switch1 : Switch  Threshold=0.5  SaturateOnIntegerOverflow=off  InputSameDT=off
  wheel-- : Outport
  wires:
  Switch1/1 -> Product2/2
  Constant3/1 -> Switch1/3
  Constant2/1 -> Switch1/1
  10/1 -> Memory3/1, Relational Operator1/1
  Relational Operator1/1 -> Switch1/2
  Memory3/1 -> Relational Operator1/2
  Memory1/1 -> Product2/1
  Product2/1 -> Product1/3, Memory1/1
  Product1/1 -> wheel--/1
  Switch/1 -> Product/2
  Constant1/1 -> Switch/3
  Constant/1 -> Switch/1
  0.1/1 -> Relational Operator2/1, Memory5/1
  Relational Operator2/1 -> Switch/2
  Memory5/1 -> Relational Operator2/2
  Memory4/1 -> Product/1
  Product/1 -> Product1/1, Memory4/1
  Data Type Conversion1/1 -> Gain/1
  Relational Operator/1 -> Data Type Conversion1/1
  Sub/1 -> Memory2/1, Relational Operator/1
  Memory2/1 -> Relational Operator/2
  Gain/1 -> Product1/2

== system EMT_ML.before_diagnostic_fixes/Power Coupler /Z1/Z/Power/Speed Sensor ==
  Ideal Rotational Motion Sensor : fl_lib/Mechanical/Mechanical Sensors/Ideal Rotational Motion Sensor  reference=foundation.enum.MeasurementReference.difference  acceleration_port=false  velocity_port=true  position_port=true  wrap_angle=false  offset=0 rad
  PS-Simulink Converter : nesl_utility/PS-Simulink Converter  PhysicalDomain=network_engine_domain  SubClassName=ps_output  LeftPortType=input  RightPortType=output  PseudoPeriodic=off  Frequencies=[]  VectorFormat=1-D array  Unit=rad/s  AffineConversion=off
  Reference : fl_lib/Mechanical/Rotational Elements/Mechanical Rotational Reference
  Tire Radius2 : Gain  Gain=30/pi
  shaft : PMIOPort  Side=Left
  r/min : Outport
  wires:
  Tire Radius2/1 -> r/min/1
  PS-Simulink Converter/1 -> Tire Radius2/1
  connections:
  shaft/RConn1 -- Ideal Rotational Motion Sensor/LConn1
  Reference/LConn1 -- Ideal Rotational Motion Sensor/RConn1
  PS-Simulink Converter/LConn1 -- Ideal Rotational Motion Sensor/RConn2

== system EMT_ML.before_diagnostic_fixes/Power Coupler /Z1/Z/Power/Torque Sensor ==
  Ideal Torque Sensor : fl_lib/Mechanical/Mechanical Sensors/Ideal Torque Sensor
  PS-Simulink Converter : nesl_utility/PS-Simulink Converter  PhysicalDomain=network_engine_domain  SubClassName=ps_output  LeftPortType=input  RightPortType=output  PseudoPeriodic=off  Frequencies=[]  VectorFormat=1-D array  Unit=1  AffineConversion=off
  In : PMIOPort  Side=Left
  Out : PMIOPort  Port=2  Side=Right
  Nm : Outport
  wires:
  PS-Simulink Converter/1 -> Nm/1
  connections:
  PS-Simulink Converter/LConn1 -- Ideal Torque Sensor/RConn2
  In/RConn1 -- Ideal Torque Sensor/LConn1
  Ideal Torque Sensor/RConn1 -- Out/RConn1

== system EMT_ML.before_diagnostic_fixes/Power Coupler /Z1/Z/Power1/Speed Sensor ==
  Ideal Rotational Motion Sensor : fl_lib/Mechanical/Mechanical Sensors/Ideal Rotational Motion Sensor  reference=foundation.enum.MeasurementReference.difference  acceleration_port=false  velocity_port=true  position_port=true  wrap_angle=false  offset=0 rad
  PS-Simulink Converter : nesl_utility/PS-Simulink Converter  PhysicalDomain=network_engine_domain  SubClassName=ps_output  LeftPortType=input  RightPortType=output  PseudoPeriodic=off  Frequencies=[]  VectorFormat=1-D array  Unit=rad/s  AffineConversion=off
  Reference : fl_lib/Mechanical/Rotational Elements/Mechanical Rotational Reference
  Tire Radius2 : Gain  Gain=30/pi
  shaft : PMIOPort  Side=Left
  r/min : Outport
  wires:
  PS-Simulink Converter/1 -> Tire Radius2/1
  Tire Radius2/1 -> r/min/1
  connections:
  PS-Simulink Converter/LConn1 -- Ideal Rotational Motion Sensor/RConn2
  Reference/LConn1 -- Ideal Rotational Motion Sensor/RConn1
  shaft/RConn1 -- Ideal Rotational Motion Sensor/LConn1

== system EMT_ML.before_diagnostic_fixes/Power Coupler /Z1/Z/Power1/Torque Sensor ==
  Ideal Torque Sensor : fl_lib/Mechanical/Mechanical Sensors/Ideal Torque Sensor
  PS-Simulink Converter : nesl_utility/PS-Simulink Converter  PhysicalDomain=network_engine_domain  SubClassName=ps_output  LeftPortType=input  RightPortType=output  PseudoPeriodic=off  Frequencies=[]  VectorFormat=1-D array  Unit=1  AffineConversion=off
  In : PMIOPort  Side=Left
  Out : PMIOPort  Port=2  Side=Right
  Nm : Outport
  wires:
  PS-Simulink Converter/1 -> Nm/1
  connections:
  Ideal Torque Sensor/RConn1 -- Out/RConn1
  In/RConn1 -- Ideal Torque Sensor/LConn1
  PS-Simulink Converter/LConn1 -- Ideal Torque Sensor/RConn2

== system EMT_ML.before_diagnostic_fixes/Power Coupler /Z1/Z/Z1/Slip Sensor ==
  Abs : Abs  SaturateOnIntegerOverflow=off
  Ideal Rotational Motion Sensor : fl_lib/Mechanical/Mechanical Sensors/Ideal Rotational Motion Sensor  reference=foundation.enum.MeasurementReference.difference  acceleration_port=false  velocity_port=true  position_port=true  wrap_angle=false  offset=0 rad
  PS-Simulink Converter : nesl_utility/PS-Simulink Converter  PhysicalDomain=network_engine_domain  SubClassName=ps_output  LeftPortType=input  RightPortType=output  PseudoPeriodic=off  Frequencies=[]  VectorFormat=1-D array  Unit=1  AffineConversion=off
  Tire Radius2 : Gain  Gain=30/pi
  In : PMIOPort  Side=Left
  Out : PMIOPort  Port=2  Side=Right
  r/min : Outport
  wires:
  PS-Simulink Converter/1 -> Tire Radius2/1
  Tire Radius2/1 -> Abs/1
  Abs/1 -> r/min/1
  connections:
  PS-Simulink Converter/LConn1 -- Ideal Rotational Motion Sensor/RConn2
  Out/RConn1 -- Ideal Rotational Motion Sensor/RConn1
  In/RConn1 -- Ideal Rotational Motion Sensor/LConn1

== system EMT_ML.before_diagnostic_fixes/Power Coupler /Z2/Z/Power/Speed Sensor ==
  Ideal Rotational Motion Sensor : fl_lib/Mechanical/Mechanical Sensors/Ideal Rotational Motion Sensor  reference=foundation.enum.MeasurementReference.difference  acceleration_port=false  velocity_port=true  position_port=true  wrap_angle=false  offset=0 rad
  PS-Simulink Converter : nesl_utility/PS-Simulink Converter  PhysicalDomain=network_engine_domain  SubClassName=ps_output  LeftPortType=input  RightPortType=output  PseudoPeriodic=off  Frequencies=[]  VectorFormat=1-D array  Unit=rad/s  AffineConversion=off
  Reference : fl_lib/Mechanical/Rotational Elements/Mechanical Rotational Reference
  Tire Radius2 : Gain  Gain=30/pi
  shaft : PMIOPort  Side=Left
  r/min : Outport
  wires:
  Tire Radius2/1 -> r/min/1
  PS-Simulink Converter/1 -> Tire Radius2/1
  connections:
  shaft/RConn1 -- Ideal Rotational Motion Sensor/LConn1
  Reference/LConn1 -- Ideal Rotational Motion Sensor/RConn1
  PS-Simulink Converter/LConn1 -- Ideal Rotational Motion Sensor/RConn2

== system EMT_ML.before_diagnostic_fixes/Power Coupler /Z2/Z/Power/Torque Sensor ==
  Ideal Torque Sensor : fl_lib/Mechanical/Mechanical Sensors/Ideal Torque Sensor
  PS-Simulink Converter : nesl_utility/PS-Simulink Converter  PhysicalDomain=network_engine_domain  SubClassName=ps_output  LeftPortType=input  RightPortType=output  PseudoPeriodic=off  Frequencies=[]  VectorFormat=1-D array  Unit=1  AffineConversion=off
  In : PMIOPort  Side=Left
  Out : PMIOPort  Port=2  Side=Right
  Nm : Outport
  wires:
  PS-Simulink Converter/1 -> Nm/1
  connections:
  PS-Simulink Converter/LConn1 -- Ideal Torque Sensor/RConn2
  In/RConn1 -- Ideal Torque Sensor/LConn1
  Ideal Torque Sensor/RConn1 -- Out/RConn1

== system EMT_ML.before_diagnostic_fixes/Power Coupler /Z2/Z/Power1/Speed Sensor ==
  Ideal Rotational Motion Sensor : fl_lib/Mechanical/Mechanical Sensors/Ideal Rotational Motion Sensor  reference=foundation.enum.MeasurementReference.difference  acceleration_port=false  velocity_port=true  position_port=true  wrap_angle=false  offset=0 rad
  PS-Simulink Converter : nesl_utility/PS-Simulink Converter  PhysicalDomain=network_engine_domain  SubClassName=ps_output  LeftPortType=input  RightPortType=output  PseudoPeriodic=off  Frequencies=[]  VectorFormat=1-D array  Unit=rad/s  AffineConversion=off
  Reference : fl_lib/Mechanical/Rotational Elements/Mechanical Rotational Reference
  Tire Radius2 : Gain  Gain=30/pi
  shaft : PMIOPort  Side=Left
  r/min : Outport
  wires:
  PS-Simulink Converter/1 -> Tire Radius2/1
  Tire Radius2/1 -> r/min/1
  connections:
  PS-Simulink Converter/LConn1 -- Ideal Rotational Motion Sensor/RConn2
  Reference/LConn1 -- Ideal Rotational Motion Sensor/RConn1
  shaft/RConn1 -- Ideal Rotational Motion Sensor/LConn1

== system EMT_ML.before_diagnostic_fixes/Power Coupler /Z2/Z/Power1/Torque Sensor ==
  Ideal Torque Sensor : fl_lib/Mechanical/Mechanical Sensors/Ideal Torque Sensor
  PS-Simulink Converter : nesl_utility/PS-Simulink Converter  PhysicalDomain=network_engine_domain  SubClassName=ps_output  LeftPortType=input  RightPortType=output  PseudoPeriodic=off  Frequencies=[]  VectorFormat=1-D array  Unit=1  AffineConversion=off
  In : PMIOPort  Side=Left
  Out : PMIOPort  Port=2  Side=Right
  Nm : Outport
  wires:
  PS-Simulink Converter/1 -> Nm/1
  connections:
  Ideal Torque Sensor/RConn1 -- Out/RConn1
  In/RConn1 -- Ideal Torque Sensor/LConn1
  PS-Simulink Converter/LConn1 -- Ideal Torque Sensor/RConn2

== system EMT_ML.before_diagnostic_fixes/Power Coupler /Z2/Z/Z2/Slip Sensor ==
  Abs : Abs  SaturateOnIntegerOverflow=off
  Ideal Rotational Motion Sensor : fl_lib/Mechanical/Mechanical Sensors/Ideal Rotational Motion Sensor  reference=foundation.enum.MeasurementReference.difference  acceleration_port=false  velocity_port=true  position_port=true  wrap_angle=false  offset=0 rad
  PS-Simulink Converter : nesl_utility/PS-Simulink Converter  PhysicalDomain=network_engine_domain  SubClassName=ps_output  LeftPortType=input  RightPortType=output  PseudoPeriodic=off  Frequencies=[]  VectorFormat=1-D array  Unit=1  AffineConversion=off
  Tire Radius2 : Gain  Gain=30/pi
  In : PMIOPort  Side=Left
  Out : PMIOPort  Port=2  Side=Right
  r/min : Outport
  wires:
  PS-Simulink Converter/1 -> Tire Radius2/1
  Tire Radius2/1 -> Abs/1
  Abs/1 -> r/min/1
  connections:
  PS-Simulink Converter/LConn1 -- Ideal Rotational Motion Sensor/RConn2
  Out/RConn1 -- Ideal Rotational Motion Sensor/RConn1
  In/RConn1 -- Ideal Rotational Motion Sensor/LConn1

== system EMT_ML.before_diagnostic_fixes/motorA/Motor/Mechanical Body/Resistance/Torque Actuator ==
  torque : Inport
  Ideal Torque Source : fl_lib/Mechanical/Mechanical Sources/Ideal Torque Source
  Mechanical Rotational Reference : fl_lib/Mechanical/Rotational Elements/Mechanical Rotational Reference
  Simulink-PS Converter : nesl_utility/Simulink-PS Converter  PhysicalDomain=network_engine_domain  SubClassName=ps_input  LeftPortType=input  RightPortType=output  PseudoPeriodic=off  Frequencies=[]  NoiseDistribution=none  NoiseParameters=[]  Unit=N*m  AffineConversion=off  FilteringAndDerivatives=zero  SimscapeFilterOrder=1  InputFilterTimeConstant=.001  UdotUserProvided=0
  shaft : PMIOPort  Side=Right
  wires:
  torque/1 -> Simulink-PS Converter/1
  connections:
  shaft/RConn1 -- Ideal Torque Source/LConn1
  Mechanical Rotational Reference/LConn1 -- Ideal Torque Source/RConn2
  Simulink-PS Converter/RConn1 -- Ideal Torque Source/RConn1

== system EMT_ML.before_diagnostic_fixes/motorB/Motor/Mechanical Body/Resistance/Torque Actuator ==
  torque : Inport
  Ideal Torque Source : fl_lib/Mechanical/Mechanical Sources/Ideal Torque Source
  Mechanical Rotational Reference : fl_lib/Mechanical/Rotational Elements/Mechanical Rotational Reference
  Simulink-PS Converter : nesl_utility/Simulink-PS Converter  PhysicalDomain=network_engine_domain  SubClassName=ps_input  LeftPortType=input  RightPortType=output  PseudoPeriodic=off  Frequencies=[]  NoiseDistribution=none  NoiseParameters=[]  Unit=N*m  AffineConversion=off  FilteringAndDerivatives=filter  SimscapeFilterOrder=1  InputFilterTimeConstant=.001  UdotUserProvided=1
  shaft : PMIOPort  Side=Right
  wires:
  torque/1 -> Simulink-PS Converter/1
  connections:
  shaft/RConn1 -- Ideal Torque Source/LConn1
  Mechanical Rotational Reference/LConn1 -- Ideal Torque Source/RConn2
  Simulink-PS Converter/RConn1 -- Ideal Torque Source/RConn1

== system EMT_ML.before_diagnostic_fixes/Control Unit/Control/Power Distribution/Feasible Control Range/State Calculation/Speed ==
  stage : Inport
  ne : Inport  Port=2
  no : Inport  Port=3
  Demux1 : Demux  Outputs=2
  Z : Subsystem
  nA : Outport
  nB : Outport  Port=2
  wires:
  Demux1/2 -> nB/1
  Demux1/1 -> nA/1
  stage/1 -> Z/1(s)
  ne/1 -> Z/2(ne)
  no/1 -> Z/3(no)
  Z/1(nAnB) -> Demux1/1

== system EMT_ML.before_diagnostic_fixes/Control Unit/Control/Power Distribution/Feasible Control Range/State Calculation/Subsystem3 ==
  0 : Inport
  Constant : Constant
  Constant1 : Constant  Value=4
  MinMax : MinMax  Function=max  Inputs=2
  MinMax1 : MinMax  Inputs=2
  1 : Outport
  wires:
  0/1 -> MinMax/1
  Constant/1 -> MinMax/2
  MinMax/1 -> MinMax1/1
  Constant1/1 -> MinMax1/2
  MinMax1/1 -> 1/1

== system EMT_ML.before_diagnostic_fixes/Control Unit/Control/Power Distribution/Feasible Control Range/State Predition/TA Range ==
  nA : Inport
  Lookup Table : Lookup  InputValues=nA_map  Table=TA_max_map  SaturateOnIntegerOverflow=off
  Lookup Table1 : Lookup  InputValues=nA_map  Table=TA_min_map  SaturateOnIntegerOverflow=off
  Mux1 : Mux  Inputs=2
  Saturation1 : Saturate  UpperLimit=max(nA_map)  LowerLimit=min(nA_map)
  Saturation2 : Saturate  UpperLimit=max(nA_map)  LowerLimit=min(nA_map)
  TA_R : Outport
  wires:
  Mux1/1 -> TA_R/1
  Saturation2/1 -> Lookup Table1/1
  Saturation1/1 -> Lookup Table/1
  Lookup Table1/1 -> Mux1/2  "TA_min"
  Lookup Table/1 -> Mux1/1  "TA_max"
  nA/1 -> Saturation1/1, Saturation2/1

== system EMT_ML.before_diagnostic_fixes/Control Unit/Control/Power Distribution/Feasible Control Range/State Predition/TB Range ==
  nB : Inport
  Lookup Table : Lookup  InputValues=nB_map  Table=TB_max_map  SaturateOnIntegerOverflow=off
  Lookup Table1 : Lookup  InputValues=nB_map  Table=TB_min_map  SaturateOnIntegerOverflow=off
  Mux1 : Mux  Inputs=2
  Saturation1 : Saturate  UpperLimit=max(nB_map)  LowerLimit=min(nB_map)
  Saturation2 : Saturate  UpperLimit=max(nB_map)  LowerLimit=min(nB_map)
  TB_R : Outport
  wires:
  Mux1/1 -> TB_R/1
  Lookup Table1/1 -> Mux1/2  "TB_min"
  Lookup Table/1 -> Mux1/1  "TB_max"
  nB/1 -> Saturation2/1, Saturation1/1
  Saturation1/1 -> Lookup Table/1
  Saturation2/1 -> Lookup Table1/1

== system EMT_ML.before_diagnostic_fixes/Control Unit/Control/Power Distribution/Feasible Control Range/State Predition/Te Range ==
  ne_act : Inport
  Constant : Constant  Value=0
  Lookup Table : Lookup  InputValues=ne_map  Table=Te_max_map  SaturateOnIntegerOverflow=off
  Mux1 : Mux  Inputs=2
  Saturation1 : Saturate  UpperLimit=max(ne_map)  LowerLimit=min(ne_map)
  Te_k : Outport
  wires:
  Mux1/1 -> Te_k/1
  ne_act/1 -> Saturation1/1
  Saturation1/1 -> Lookup Table/1
  Constant/1 -> Mux1/2  "Te_min"
  Lookup Table/1 -> Mux1/1  "Te_max"

== system EMT_ML.before_diagnostic_fixes/Control Unit/Control/Power Distribution/Feasible Control Range/State Predition/Z ==
  stage : Inport
  ne_act : Inport  Port=2
  no_act : Inport  Port=3
  Mux2 : Mux  Inputs=3
  Saturation1 : Saturate  UpperLimit=ne_max  LowerLimit=ne_min
  Saturation2 : Saturate  UpperLimit=ne_max  LowerLimit=ne_min
  ne Range : Subsystem
  ne_k : Outport
  wires:
  Saturation2/1 -> Mux2/3
  Saturation1/1 -> Mux2/2
  ne_act/1 -> Mux2/1
  ne Range/1(ne_max) -> Saturation1/1
  ne Range/2(ne_min) -> Saturation2/1
  Mux2/1 -> ne_k/1
  stage/1 -> ne Range/1(stage)
  no_act/1 -> ne Range/2(no)

== system EMT_ML.before_diagnostic_fixes/Control Unit/Control/Prepare Stage/motorA torque/TA_com1/Subsystem1 ==
  nA_act : Inport
  Constant : Constant  Value=a11*(ne_idl+100)
  StartupFeedbackDelay : TransportDelay  DelayTime=startup_feedback_delay_s
  Subsystem : Subsystem
  Sum1 : Sum  Inputs=+-
  TA_com : Outport
  wires:
  Subsystem/1(TA) -> TA_com/1
  StartupFeedbackDelay/1 -> Sum1/2
  nA_act/1 -> StartupFeedbackDelay/1
  Sum1/1 -> Subsystem/1(dnA)
  Constant/1 -> Sum1/1

== system EMT_ML.before_diagnostic_fixes/Control Unit/Control/Prepare Stage/motorA torque/TA_com1/Subsystem2 ==
  PN : Inport
  nA : Inport  Port=2
  Fcn : Fcn  Expr=9549*(u(1)+abs(u(1)))/2*startup_power_share/sqrt(u(2)^2+startup_speed_regularizer_rpm^2)*(1-TS_A*u(2)*u(3)/(u(2)^2+startup_speed_regularizer_rpm^2))
  Mux : Mux  Inputs=3
  StartupGovernorLog : ToWorkspace  VariableName=startup_governor_trace  SaveFormat=Structure With Time  SampleTime=-1
  StartupGovernorTrace : Mux  Inputs=2
  StartupSpeedDerivative : Derivative
  TA_com : Outport
  wires:
  StartupGovernorTrace/1 -> StartupGovernorLog/1
  StartupSpeedDerivative/1 -> Mux/3
  nA/1 -> StartupSpeedDerivative/1, Mux/2
  Fcn/1 -> StartupGovernorTrace/2, TA_com/1
  PN/1 -> Mux/1
  Mux/1 -> StartupGovernorTrace/1, Fcn/1

== system EMT_ML.before_diagnostic_fixes/Control Unit/Control/Shift Stage/EVT2->EVT1/motorZ torque/Subsystem1 ==
  nZ_act : Inport
  Constant3 : Constant  Value=0
  Memory5 : Memory
  PID Controller2 : simulink_need_slupdate/PID Controller  P=2  I=0.01  D=0.1
  Sum1 : Sum  Inputs=+-
  TZ_com : Outport
  wires:
  Memory5/1 -> Sum1/2
  Constant3/1 -> Sum1/1
  nZ_act/1 -> Memory5/1
  Sum1/1 -> PID Controller2/1
  PID Controller2/1 -> TZ_com/1
